simulink model "test_SimulinkMdl3LPV_MPC_a"  (R2019b)
settings: Solver=FixedStepAuto  StartTime=0.0  StopTime=400  FixedStep=DT  RelTol=1e-3
values from neighbouring files (symbols this model uses):
  DT = 0.008    [dataDLR.m]    (also in generateReport.m; initLPVParam.m; initWorkspace.m; runCalculateEvalCriteria.m)
  Lin_points : value not decoded    [DD_test.sldd]
undefined symbols (not defined in the file or in its folder): Rotor_Lambda
settings Model: DataDictionary=DD_test.sldd  ExtModeTrigMode=oneshot  ExtModeArmWhenConnect=off  Creator=Hazim Namik  LastModifiedBy=ditt_aj
settings DataIOCC: LimitDataPoints=on  SaveFormat=Array  ReturnWorkspaceOutputs=off
settings OptimizationCC: BlockReduction=off  BooleanDataType=off  LifeSpan=inf
settings DebuggingCC: SaveWithParameterizedLinksMsg=none  UnderspecifiedInitializationDetection=Classic  MergeDetectMultiDrivingBlocksExec=none  SignalResolutionControl=TryResolveAllWithWarning  SFUnexpectedBacktrackingDiag=warning  SFNoUnconditionalDefaultTransitionDiag=warning  SFExecutionAtInitializationDiag=none  ArithmeticOperatorsInVariantConditions=warning
settings HardwareCC: ProdBitPerPointer=32  ProdBitPerSizeT=32  ProdBitPerPtrDiffT=32  ProdLargestAtomicFloat=None  ProdIntDivRoundTo=Undefined  ProdEndianess=Unspecified  ProdWordSize=32  ProdHWDeviceType=32-bit Generic  TargetUnknown=on
settings ModelReferenceCC: PropagateSignalLabelsOutOfModel=off
settings SFSimCC: SimUseLocalCustomCode=off  CustomCodeUndefinedFunction=UseInterfaceOnly
settings RTWCC: RTWUseLocalCustomCode=off
settings CodeAppCC: StateflowObjectComments=on
settings GRTTargetCC: TargetLangStandard=C89/C90 (ANSI)  GeneratePreprocessorConditionals=Disable all
settings ConfigComp: CovMetricSettings=dw  CovHtmlReporting=on  CovSaveCumulativeToWorkspaceVar=on  CovSaveSingleToWorkspaceVar=on  CovExternalEMLEnable=off

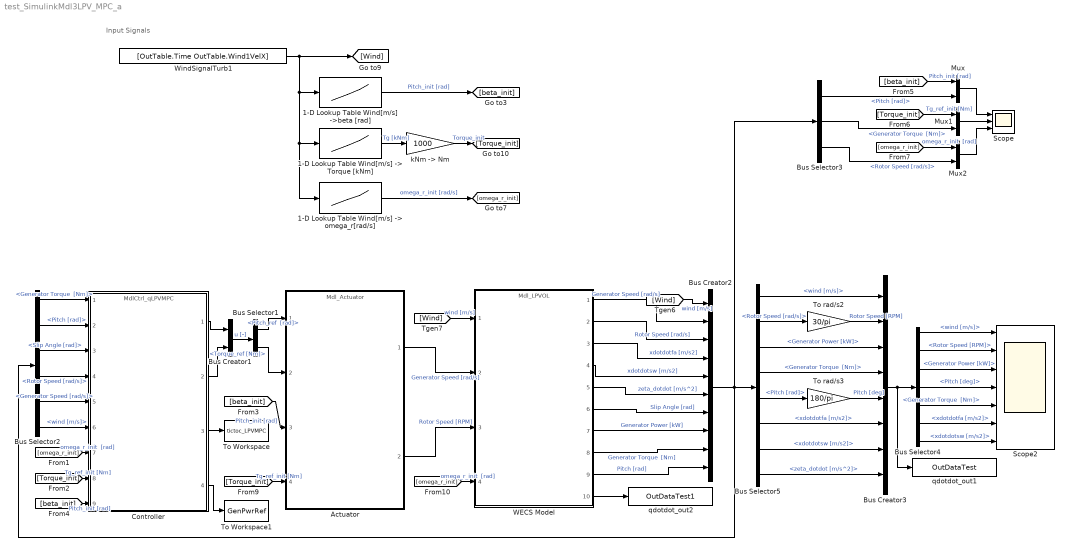
== system test_SimulinkMdl3LPV_MPC_a ==
  note: Input Signals
  "1-D Lookup Table Wind[m/s] -> Torque [kNm]" : Lookup_n-D  NumberOfTableDimensions=1  BreakpointsForDimension1=Lin_points.V  BreakpointsForDimension2=Rotor_Lambda  Table=Lin_points.Torque  InternalRulePriority=Speed  RndMeth=Simplest  InputSameDT=on
  "1-D Lookup Table Wind[m/s] -> omega_r[rad/s]" : Lookup_n-D  NumberOfTableDimensions=1  BreakpointsForDimension1=Lin_points.V  BreakpointsForDimension2=Rotor_Lambda  Table=Lin_points.RSpeed  InternalRulePriority=Speed  RndMeth=Simplest  InputSameDT=on
  1-D Lookup Table Wind[m/s] ->beta [rad] : Lookup_n-D  NumberOfTableDimensions=1  BreakpointsForDimension1=Lin_points.V  BreakpointsForDimension2=Rotor_Lambda  Table=Lin_points.Pitch  InternalRulePriority=Speed  RndMeth=Simplest  InputSameDT=on
  Actuator : ModelReference  ModelNameDialog=Mdl_Actuator.slx  SimulationMode=Normal  ModelReferenceVersion=1.7
  Bus Creator1 : BusCreator  Inputs=2
  Bus Creator2 : BusCreator  Inputs=10
  Bus Creator3 : BusCreator  Inputs=8
  Bus Selector1 : BusSelector  OutputSignals="Pitch_ref  [rad],Torque_ref [Nm]"
  Bus Selector2 : BusSelector  OutputSignals="Generator Torque  [Nm],Pitch [rad],Slip Angle [rad],Rotor Speed [rad/s],Generator Speed [rad/s],wind [m/s]"
  Bus Selector3 : BusSelector  OutputSignals="Pitch [rad],Generator Torque  [Nm],Rotor Speed [rad/s]"
  Bus Selector4 : BusSelector  OutputSignals="wind [m/s],Rotor Speed [RPM],Generator Power [kW],Pitch [deg],Generator Torque  [Nm],xdotdotfa [m/s2],xdotdotsw [m/s2]"
  Bus Selector5 : BusSelector  OutputSignals="wind [m/s],Rotor Speed [rad/s],Generator Power [kW],Generator Torque  [Nm],Pitch [rad],xdotdotfa [m/s2],xdotdotsw [m/s2],zeta_dotdot [m/s^2]"
  Controller : ModelReference  ModelNameDialog=MdlCtrl_qLPVMPC.slx  SimulationMode=Normal  ModelReferenceVersion=1.29
  Mux : Mux  Inputs=2
  Mux1 : Mux  Inputs=2
  Mux2 : Mux  Inputs=2
  Scope : Scope  NumInputPorts=3
  Scope2 : Scope  NumInputPorts=7
      settings: Tag=Scope
  To Workspace : ToWorkspace  VariableName=tictoc_LPVMPC  SaveFormat=Timeseries  SampleTime=-1
  To Workspace1 : ToWorkspace  VariableName=GenPwrRef  SaveFormat=Timeseries  SampleTime=-1
  To rad/s2 : Gain  Gain=30/pi
  To rad/s3 : Gain  Gain=180/pi
  WECS Model : ModelReference  ModelNameDialog=Mdl_LPVOL.slx  SimulationMode=Normal  ModelReferenceVersion=1.55
  WindSignalTurb1 : FromWorkspace  VariableName=[OutTable.Time OutTable.Wind1VelX]  SampleTime=DT  OutputAfterFinalValue=Holding final value
  "kNm -> Nm" : Gain  Gain=1000
  qdotdot_out1 : ToWorkspace  VariableName=OutDataTest  SampleTime=-1
  qdotdot_out2 : ToWorkspace  VariableName=OutDataTest1  SampleTime=-1
  wires:
  Bus Creator1/1 -> Bus Selector1/1  "u [-]"
  [omega_r_init] -> Controller/7  "omega_r_init  [rad]"
  Bus Selector1/2 -> Actuator/2  "<Torque_ref [Nm]>"
  [beta_init] -> Controller/9  "Pitch_init [rad]"
  WindSignalTurb1/1 -> [Wind], "1-D Lookup Table Wind[m/s] -> omega_r[rad/s]"/1, "1-D Lookup Table Wind[m/s] -> Torque [kNm]"/1, 1-D Lookup Table Wind[m/s] ->beta [rad]/1
  Bus Selector2/4 -> Controller/4  "<Rotor Speed [rad/s]>"
  "kNm -> Nm"/1 -> [Torque_init]  "Torque_init"
  Controller/1 -> Bus Creator1/1
  Controller/3 -> To Workspace/1
  Actuator/2 -> WECS Model/3  "Rotor Speed [RPM]"
  Bus Selector2/3 -> Controller/3  "<Slip Angle [rad]>"
  Controller/2 -> Bus Creator1/2
  Bus Selector2/2 -> Controller/2  "<Pitch [rad]>"
  [Torque_init] -> Controller/8  "Tg_ref_init [Nm]"
  Bus Selector2/6 -> Controller/6  "<wind [m/s]>"
  [beta_init] -> Actuator/3  "Pitch_init [rad]"
  "1-D Lookup Table Wind[m/s] -> omega_r[rad/s]"/1 -> [omega_r_init]  "omega_r_init [rad/s]"
  Bus Selector1/1 -> Actuator/1  "<Pitch_ref  [rad]>"
  [Wind] -> WECS Model/1  "wind [m/s]"
  1-D Lookup Table Wind[m/s] ->beta [rad]/1 -> [beta_init]  "Pitch_init [rad]"
  "1-D Lookup Table Wind[m/s] -> Torque [kNm]"/1 -> "kNm -> Nm"/1  "Tg [kNm]"
  Bus Selector2/5 -> Controller/5  "<Generator Speed [rad/s]>"
  Bus Selector2/1 -> Controller/1  "<Generator Torque  [Nm]>"
  [Torque_init] -> Actuator/4  "Tg_ref_init [Nm]"
  Actuator/1 -> WECS Model/2  "Generator Speed [rad/s]"
  [omega_r_init] -> WECS Model/4  "omega_r_init  [rad]"
  Controller/4 -> To Workspace1/1
  WECS Model/8 -> Bus Creator2/9  "Generator Torque  [Nm]"
  WECS Model/7 -> Bus Creator2/8  "Generator Power [kW]"
  WECS Model/2 -> Bus Creator2/3  "Rotor Speed [rad/s]"
  WECS Model/4 -> Bus Creator2/5  "xdotdotsw [m/s2]"
  WECS Model/3 -> Bus Creator2/4  "xdotdotfa [m/s2]"
  WECS Model/1 -> Bus Creator2/2  "Generator Speed [rad/s]"
  WECS Model/5 -> Bus Creator2/6  "zeta_dotdot [m/s^2]"
  WECS Model/9 -> Bus Creator2/10  "Pitch [rad]"
  [Wind] -> Bus Creator2/1  "wind [m/s]"
  WECS Model/6 -> Bus Creator2/7  "Slip Angle [rad]"
  Bus Selector5/8 -> Bus Creator3/8  "<zeta_dotdot [m/s^2]>"
  Bus Selector4/3 -> Scope2/3  "<Generator Power [kW]>"
  Bus Selector4/6 -> Scope2/6  "<xdotdotfa [m/s2]>"
  Bus Creator3/1 -> Bus Selector4/1, qdotdot_out1/1
  Bus Selector4/7 -> Scope2/7  "<xdotdotsw [m/s2]>"
  To rad/s3/1 -> Bus Creator3/5  "Pitch [deg]"
  Bus Selector5/3 -> Bus Creator3/3  "<Generator Power [kW]>"
  Bus Selector5/2 -> To rad/s2/1  "<Rotor Speed [rad/s]>"
  Bus Selector4/1 -> Scope2/1  "<wind [m/s]>"
  Bus Selector4/2 -> Scope2/2  "<Rotor Speed [RPM]>"
  Bus Selector4/4 -> Scope2/4  "<Pitch [deg]>"
  Bus Selector4/5 -> Scope2/5  "<Generator Torque  [Nm]>"
  Bus Selector5/5 -> To rad/s3/1  "<Pitch [rad]>"
  Bus Selector5/1 -> Bus Creator3/1  "<wind [m/s]>"
  To rad/s2/1 -> Bus Creator3/2  "Rotor Speed [RPM]"
  Bus Selector5/4 -> Bus Creator3/4  "<Generator Torque  [Nm]>"
  Bus Selector5/7 -> Bus Creator3/7  "<xdotdotsw [m/s2]>"
  Bus Selector5/6 -> Bus Creator3/6  "<xdotdotfa [m/s2]>"
  [omega_r_init] -> Mux2/1  "omega_r_init  [rad]"
  Mux1/1 -> Scope/2
  Bus Selector3/1 -> Mux/2  "<Pitch [rad]>"
  Bus Creator2/1 -> Bus Selector2/1, Bus Selector3/1, Bus Selector5/1
  [beta_init] -> Mux/1  "Pitch_init [rad]"
  Bus Selector3/2 -> Mux1/2  "<Generator Torque  [Nm]>"
  Mux/1 -> Scope/1
  Bus Selector3/3 -> Mux2/2  "<Rotor Speed [rad/s]>"
  [Torque_init] -> Mux1/1  "Tg_ref_init [Nm]"
  Mux2/1 -> Scope/3
  WECS Model/10 -> qdotdot_out2/1
